simulink library "ConverterLibrary"  (R2026a)
settings: Solver=VariableStepAuto
undefined symbols (not defined in the file or in its folder): DiscIntNeverNeededParam, dspblkCoreblockFVToolHelper, gcbh, gridInverter
libraries: fl_lib x240, nesl_utility x221, ee_lib x208, slpidlib x28, eeGeneralControl x12, simulink x9, eeTransforms x4, simulink_extras x1, eePowerMeasurement x1
(part 1 of 30)
settings Model: Creator=vsolaise  LastModifiedBy=vsolaise

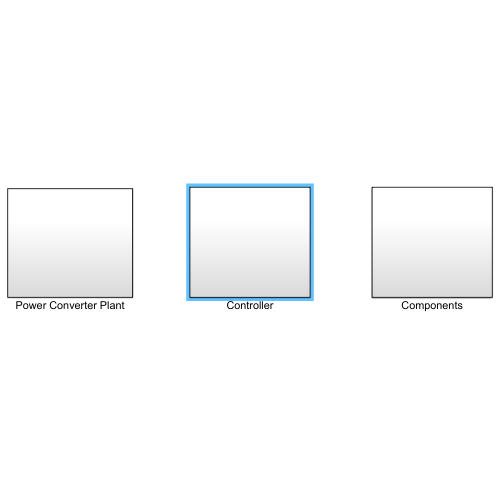
[thumbnail: Simulink's stored preview of the top-level diagram]
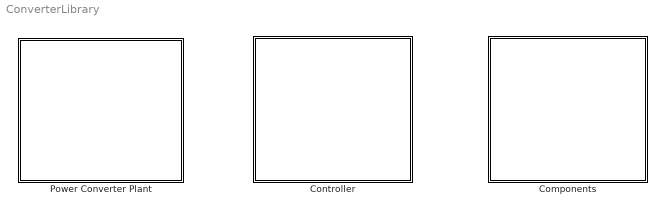
== system ConverterLibrary ==
  Components : Subsystem
  Controller : Subsystem
  Power Converter Plant : Subsystem

== system ConverterLibrary/Components ==
  Diode Model : Subsystem  mask(Diode thermal model){Tj_diode=[25, 125]+273.15, Tj_diode_unit=K, If_data=[.1, .2, .5, 1, 2, 4, 7, 10], If_data_unit=A, Vf_data=[.9, 1.15, 1.25, 1.5, 1.75, 2.17, 2.6, 2.85; .58, .68, .75, 1.1, 1.38, 1.77, 2.27, 2.7], Vf_data_unit=V, thermal_resistance=0.3, thermal_resistance_unit=K/W, thermal_mass=0.001, thermal_mass_unit=J/K, Tj0=300, Tj0_unit=K, diodeVf=0.8, diodeVf_unit=V, diodeRon=0.001, diodeRon_unit=Ohm, diodeGoff=1e-5, diodeGoff_unit=1/Ohm, Recovery_Loss_Flag=on, Tj_rec=[25, 125]+273.15, Tj_rec_unit=K, If_rec_data=[.1, .2, .5, 1, 2, 4, 7, 10], If_rec_data_unit=A, Erec_data=1e-6*[0.05 0.1 0.4 1 2.6 6 11.5 17.5; 0.1 0.2 0.8 2.1 5.2 12 23 35], Erec_data_unit=J, Vrec_ref=300, Vrec_ref_unit=V, Irec_min=1e-3, Irec_min_unit=A}
      mask prompts: Tj_diode "Junction temperature vector, Tj"; If_data "Forward current vector, If"; Vf_data "Forward voltage, Vf(Tj,If)"; thermal_resistance "Junction-case resistance"; thermal_mass "Junction thermal mass"; Tj0 "Initial temperature"; diodeVf "Forward voltage, Vf"; diodeRon "On-state resistance, Ron"; diodeGoff "Off-state conductance, Goff"; Recovery_Loss_Flag "Include reverse recovery loss"; Tj_rec "Junction temperature vector, Tj"; If_rec_data "Forward current vector before commutation, If"; Erec_data "Reverse recovery energy, Erec(Tj,If)"; Vrec_ref "Voltage at which Erec was measured, Vref"; Irec_min "Forward current below which the diode counts as off"
      mask help: This block implements a diode with a thermal port using a Simulink interface for better simulation performance. The electrical model is simple-fidelity; conduction loss is evaluated from the tabulated I-V curve and reverse recovery loss from a tabulated recovery energy, both in Simulink. Together they drive the junction temperature, which is applied back to the thermal port. Ports + and - are the electrical terminals; port A is the ambient (case) thermal port.
      mask init:
      | % Unit conversion - convert to internal units: V, A, Ohm, 1/Ohm, J, K, K/W, J/K
      | 
      | % Voltage (to V)
      | if strcmp(diodeVf_unit, 'mV'), diodeVf = diodeVf / 1000; end
      | if strcmp(Vf_data_unit, 'mV'), Vf_data = Vf_data / 1000; end
      | if strcmp(Vrec_ref_unit, 'kV'), Vrec_ref = Vrec_ref * 1000; end
      | 
      | % Current (to A)
      | if strcmp(If_data_unit, 'mA'), If_data = If_data / 1000; end
      | if strcmp(If_rec_data_unit, 'mA'), If_rec_data = If_rec_data / 1000; end
      | if strcmp(Irec_min_unit, 'mA'), Irec_min = Irec_min / 1000; end
      | 
      | % Resistance and conductance (to Ohm and 1/Ohm; S is identical to 1/Ohm)
      | if strcmp(diodeRon_unit, 'mOhm'), diodeRon = diodeRon / 1000; end
      | if strcmp(diodeGoff_unit, 'mS'), diodeGoff = diodeGoff / 1000; end
      | 
      | % Energy (to J)
      | if strcmp(Erec_data_unit, 'mJ'), Erec_data = Erec_data / 1000; end
      | if strcmp(Erec_data_unit, 'uJ'), Erec_data = Erec_data / 1e6; end
      | 
      | % Temperature (to K)
      | if strcmp(Tj_diode_unit, 'degC'), Tj_diode = Tj_diode + 273.15; end
      | if strcmp(Tj_rec_unit, 'degC'), Tj_rec = Tj_rec + 273.15; end
      | if strcmp(Tj0_unit, 'degC'), Tj0 = Tj0 + 273.15; end
      | 
      | % Thermal mass (to J/K)
      | if strcmp(thermal_mass_unit, 'kJ/K'), thermal_mass = thermal_mass * 1000; end
      | 
      | % Reverse recovery on or off. Folded into the Recovery step gain, so clearing
      | % the box removes the contribution rather than scaling it by something small.
      | if strcmp(get_param(gcb, 'Recovery_Loss_Flag'), 'on')
      |     RecoveryLossFlag = 1;
      | else
      |     RecoveryLossFlag = 0;
      | end
      mask Help: web('DiodeModel.html')
      mask TypeOptions Tj_diode_unit: K | degC
      mask TypeOptions If_data_unit: A | mA
      mask TypeOptions Vf_data_unit: V | mV
      mask TypeOptions thermal_resistance_unit: K/W | degC/W
      mask TypeOptions thermal_mass_unit: J/K | kJ/K
      mask TypeOptions Tj0_unit: K | degC
      mask TypeOptions diodeVf_unit: V | mV
      mask TypeOptions diodeRon_unit: Ohm | mOhm
      mask TypeOptions diodeGoff_unit: 1/Ohm | S | mS
      mask TypeOptions Tj_rec_unit: K | degC
      mask TypeOptions If_rec_data_unit: A | mA
      mask TypeOptions Erec_data_unit: J | mJ | uJ
      mask TypeOptions Vrec_ref_unit: V | kV
      mask TypeOptions Irec_min_unit: A | mA
      mask DialogControl conduction Prompt: Diode electrical parameters
      mask DialogControl switching Prompt: Reverse recovery loss parameters
      mask DialogControl diodeConduction Prompt: Conduction loss (I-V curve)
      mask DialogControl thermal Prompt: Thermal parameters
      mask Display: image('diode_thermal.svg');
  IGBT Model : Subsystem  mask(IGBT thermal model){Vth=0.5, Vth_unit=V, Von_data=[ 0 1.1 1.3 1.45 1.75 2.25 2.7; 0 1 1.15 1.35 1.7 2.35 3 ], Von_data_unit=V, Tj=[ 298.15 398.15 ], Tj_unit=K, Iout_data=0.1*[ 0 10 50 100 200 400 600 ], Iout_data_unit=A, Iout_data_loss=0.1*[ 0 10 50 100 200 400 600 ], Iout_data_loss_unit=A, Tj_loss=[ 298.15 398.15 ], Tj_loss_unit=K, Eoff_data=0.1*[ 0 2.1e-4 1.07e-3 2.14e-3 4.29e-3 9.86e-3 1.714e-2; 0 4.3e-4 1.97e-3 3.86e-3 7.71e-3 1.543e-2 2.271e-2 ], Eoff_data_unit=J, Eon_data=0.1*[ 0 2.9e-4 1.43e-3 2.86e-3 5.71e-3 1.314e-2 2.286e-2; 0 5.7e-4 2.63e-3 5.14e-3 1.029e-2 2.057e-2 3.029e-2 ], Eon_data_unit=J, Voff=300, Voff_unit=V, Soft_Switching_Flag=on, Tj_diode=[25, 125]+273.15, Tj_diode_unit=K, If_data=[.1, .2, .5, 1, 2, 4, 7, 10], If_data_unit=A, Vf_data=[.9, 1.15, 1.25, 1.5, 1.75, 2.17, 2.6, 2.85; .58, .68, .75, 1.1, 1.38, 1.77, 2.27, 2.7], Vf_data_unit=V, thermal_resistance=0.3, thermal_resistance_unit=K/W, thermal_mass=0.001, thermal_mass_unit=J/K, Tj0=300, Tj0_unit=K, VfIGBT=0.8, VfIGBT_unit=V, Ron=0.001, Ron_unit=Ohm, Goff=1e-5, Goff_unit=1/Ohm, diodeOption=Inbuilt diode, diodeVf=0.8, diodeVf_unit=V, diodeRon=0.001, diodeRon_unit=Ohm, diodeGoff=1e-5, diodeGoff_unit=1/Ohm}
      mask prompts: Vth "Threshold voltage"; Von_data "On-state voltage, Vce(Tj,Ice)"; Tj "Temperature vector, Tj"; Iout_data "Collector-emitter current vector, Ice"; Iout_data_loss "Collector-emitter current vector, Ice"; Tj_loss "Temperature vector, Tj"; Eoff_data "Switch-off loss, Eoff(Tj,Ids)"; Eon_data "Switch-on loss, Eon(Tj,Ids)"; Voff "Off-state voltage"; Soft_Switching_Flag "Soft-Switching Application"; Tj_diode "Temperature vector"; If_data "Current vector"; Vf_data "Diode voltage, Vf(Tj,Id)"; thermal_resistance "Junction-case resistance"; thermal_mass "Junction thermal mass"; Tj0 "Initial temperature"; VfIGBT "Forward voltage, Vf"; Ron "On-state resistance, Ron"; Goff "Off-state conductance, Goff"; diodeOption "Anti-parallel diode"; diodeVf "Diode forward voltage, Vf"; diodeRon "Diode on-state resistance, Ron"; diodeGoff "Diode off-state conductance, Goff"
      mask help: This block implements the IGBT (Ideal, Switching) with a thermal port using a Simulink interface for better simulation performance. Conduction, switching and anti-parallel diode losses are evaluated in Simulink and drive the junction temperature, which is applied back to the thermal port.
      mask init:
      | % Unit conversion - convert to internal units: V, A, Ohm, 1/Ohm, J, K, K/W, J/K
      | if strcmp(Vth_unit, 'mV'), Vth = Vth / 1000; end
      | if strcmp(VfIGBT_unit, 'mV'), VfIGBT = VfIGBT / 1000; end
      | if strcmp(Ron_unit, 'mOhm'), Ron = Ron / 1000; end
      | if strcmp(Goff_unit, 'mS'), Goff = Goff / 1000; end
      | if strcmp(Von_data_unit, 'mV'), Von_data = Von_data / 1000; end
      | if strcmp(Voff_unit, 'kV'), Voff = Voff * 1000; end
      | if strcmp(diodeVf_unit, 'mV'), diodeVf = diodeVf / 1000; end
      | if strcmp(diodeRon_unit, 'mOhm'), diodeRon = diodeRon / 1000; end
      | if strcmp(diodeGoff_unit, 'mS'), diodeGoff = diodeGoff / 1000; end
      | if strcmp(Vf_data_unit, 'mV'), Vf_data = Vf_data / 1000; end
      | if strcmp(Iout_data_unit, 'mA'), Iout_data = Iout_data / 1000; end
      | if strcmp(Iout_data_loss_unit, 'mA'), Iout_data_loss = Iout_data_loss / 1000; end
      | if strcmp(If_data_unit, 'mA'), If_data = If_data / 1000; end
      | if strcmp(Eoff_data_unit, 'mJ'), Eoff_data = Eoff_data / 1000; end
      | if strcmp(Eoff_data_unit, 'uJ'), Eoff_data = Eoff_data / 1e6; end
      | if strcmp(Eon_data_unit, 'mJ'), Eon_data = Eon_data / 1000; end
      | if strcmp(Eon_data_unit, 'uJ'), Eon_data = Eon_data / 1e6; end
      | if strcmp(Tj_unit, 'degC'), Tj = Tj + 273.15; end
      | if strcmp(Tj_loss_unit, 'degC'), Tj_loss = Tj_loss + 273.15; end
      | if strcmp(Tj_diode_unit, 'degC'), Tj_diode = Tj_diode + 273.15; end
      | if strcmp(Tj0_unit, 'degC'), Tj0 = Tj0 + 273.15; end
      | if strcmp(thermal_mass_unit, 'kJ/K'), thermal_mass = thermal_mass * 1000; end
      | 
      | % Off-state leakage loss: the IGBT, plus the anti-parallel diode when it is inbuilt.
      | if strcmp(get_param(gcb, 'diodeOption'), 'Inbuilt diode')
      |     leakageConductance = Goff + diodeGoff;
      | else
      |     leakageConductance = Goff;
      | end
      | 
      | % Hard- versus soft-switching sampling, consumed inside the Thermal model.
      | currentStatus = get_param(gcb, 'Soft_Switching_Flag');
      | if strcmp(currentStatus, 'on')
      |     SwitchLossFlag = 1;
      | else
      |     SwitchLossFlag = 0;
      | end
      | 
      | % Apply the anti-parallel diode option: variant choice plus parameter visibility.
      | selectIGBTModelDiodeOption(gcb);
      mask Help: web('IGBTModel.html')
      mask TypeOptions Vth_unit: V | mV
      mask TypeOptions Von_data_unit: V | mV
      mask TypeOptions Tj_unit: K | degC
      mask TypeOptions Iout_data_unit: A | mA
      mask TypeOptions Iout_data_loss_unit: A | mA
      mask TypeOptions Tj_loss_unit: K | degC
      mask TypeOptions Eoff_data_unit: J | mJ | uJ
      mask TypeOptions Eon_data_unit: J | mJ | uJ
      mask TypeOptions Voff_unit: V | kV
      mask Callback Soft_Switching_Flag:
      | currentStatus = get_param(gcb, 'Soft_Switching_Flag');
      | if strcmp(currentStatus, 'on')
      |     SwitchLossFlag = 1;
      | else
      |     SwitchLossFlag = 0;
      | end
      mask TypeOptions Tj_diode_unit: K | degC
      mask TypeOptions If_data_unit: A | mA
      mask TypeOptions Vf_data_unit: V | mV
      mask TypeOptions thermal_resistance_unit: K/W | degC/W
      mask TypeOptions thermal_mass_unit: J/K | kJ/K
      mask TypeOptions Tj0_unit: K | degC
      mask TypeOptions VfIGBT_unit: V | mV
      mask TypeOptions Ron_unit: Ohm | mOhm
      mask TypeOptions Goff_unit: 1/Ohm | S | mS
      mask TypeOptions diodeOption: Inbuilt diode | External diode
      mask Callback diodeOption: selectIGBTModelDiodeOption(gcb);
      mask TypeOptions diodeVf_unit: V | mV
      mask TypeOptions diodeRon_unit: Ohm | mOhm
      mask TypeOptions diodeGoff_unit: 1/Ohm | S | mS
      mask DialogControl conduction Prompt: IGBT conduction parameters
      mask DialogControl switching Prompt: IGBT switching parameters
      mask DialogControl diodeConduction Prompt: Anti-parallel diode parameters
      mask DialogControl thermal Prompt: Thermal parameters
      mask Display: image('n_igbt_thermal.svg');
  MOSFET Model : Subsystem  mask(MOSFET thermal model){Vth=3.2, Vth_unit=V, Von_data=[-3.075 -1.321 -0.5334 -0.2017 -5.735e-2 0 5.654e-2 0.1988 0.6074 1.756 5.672; -4.404 -1.709 -0.657 -0.2346 -0.0667 0 6.456e-2 0.227 0.6342 1.831 6.194; -4.759 -3.111 -1.191 -0.4253 -0.1209 0 0.1049 0.369 1.1 3.268 12.47; -5.366 -4.667 -1.787 -0.638 -0.1813 0 0.1573 0.5535 1.65 4.902 18.71], Von_data_unit=V, Tj=[-55 25 150 900], Tj_unit=degC, Iout_data=[-99.94 -39.11 -14.94 -5.333 -1.517 0 1.517 5.334 14.94 39.12 99.97], Iout_data_unit=A, Iout_data_loss=[0 16.04 32.08 48.12 64.15 80.19], Iout_data_loss_unit=A, Tj_loss=[-55 25 150 900 1000], Tj_loss_unit=degC, Eoff_data=[0 1.079e-4 2.792e-4 6.058e-4 1.107e-3 1.708e-3; 0 1.046e-4 2.706e-4 5.872e-4 1.073e-3 1.655e-3; 0 1.303e-4 3.368e-4 7.31e-4 1.336e-3 2.061e-3; 0 1.433e-4 3.705e-4 8.041e-4 1.47e-3 2.267e-3; 0 1.433e-4 3.705e-4 8.041e-4 1.47e-3 2.267e-3], Eoff_data_unit=J, Eon_data=[0 2.53e-4 7.404e-4 1.481e-3 2.418e-3 3.535e-3; 0 2.341e-4 6.85e-4 1.37e-3 2.237e-3 3.27e-3; 0 2.172e-4 6.356e-4 1.272e-3 2.076e-3 3.035e-3; 0 1.955e-4 5.72e-4 1.145e-3 1.868e-3 2.732e-3; 0 1.955e-4 5.72e-4 1.145e-3 1.868e-3 2.732e-3], Eon_data_unit=J, Voff=800, Voff_unit=V, Soft_Switching_Flag=on, Tj_diode=[-55 25 150 900 1000], Tj_diode_unit=degC, If_data=[0 1.516 5.33 14.93 39.07 99.82], If_data_unit=A, Vf_data=[0 3.294 3.769 4.385 5.249 6.672; 0 2.997 3.415 3.921 4.714 5.992; 0 2.624 2.988 3.498 4.274 5.6; 0 2.362 2.689 3.148 3.847 5.04; 0 2.362 2.689 3.148 3.847 5.04], Vf_data_unit=V, thermal_resistance=0.001, thermal_resistance_unit=K/W, thermal_mass=0.01, thermal_mass_unit=J/K, Tj0=25, Tj0_unit=degC, Goff=1e-5, Goff_unit=S, Rds=0.044, Rds_unit=Ohm, GdsOff=8.3333e-13, GdsOff_unit=S}
      mask prompts: Vth "Threshold voltage"; Von_data "On-state voltage, Vdson(Tj,Ids)"; Tj "Temperature vector, Tj"; Iout_data "Drain-source vector, Ids"; Iout_data_loss "Drain-source current vector, Ids"; Tj_loss "Temperature vector, Tj"; Eoff_data "Switch-off loss, Eoff(Tj,Ids)"; Eon_data "Switch-on loss, Eon(Tj,Ids)"; Voff "Off-state voltage"; Soft_Switching_Flag "Soft-Switching Application"; Tj_diode "Temperature vector"; If_data "Current vector"; Vf_data "Diode voltage Vf(Tj,Id)"; thermal_resistance "Junction-case resistance"; thermal_mass "Junction thermal mass"; Tj0 "Initial temperature"; Goff "Diode off-state conductance"; Rds "On-state resistance"; GdsOff "Off-state conductance"
      mask help: This block implements the MOSFET (Ideal, Switching) with thermal ports using SimuLink interface for better simulation performance.
      mask init:
      | % Unit conversion - convert to internal units: V, A, J, K, K/W, J/K, S
      | 
      | % Voltage (to V)
      | if strcmp(Vth_unit, 'mV'), Vth = Vth / 1000; end
      | if strcmp(Von_data_unit, 'mV'), Von_data = Von_data / 1000; end
      | if strcmp(Voff_unit, 'kV'), Voff = Voff * 1000; end
      | if strcmp(Vf_data_unit, 'mV'), Vf_data = Vf_data / 1000; end
      | 
      | % Current (to A)
      | if strcmp(Iout_data_unit, 'mA'), Iout_data = Iout_data / 1000; end
      | if strcmp(Iout_data_loss_unit, 'mA'), Iout_data_loss = Iout_data_loss / 1000; end
      | if strcmp(If_data_unit, 'mA'), If_data = If_data / 1000; end
      | 
      | % Energy (to J)
      | if strcmp(Eoff_data_unit, 'mJ'), Eoff_data = Eoff_data / 1000; end
      | if strcmp(Eoff_data_unit, 'uJ'), Eoff_data = Eoff_data / 1e6; end
      | if strcmp(Eon_data_unit, 'mJ'), Eon_data = Eon_data / 1000; end
      | if strcmp(Eon_data_unit, 'uJ'), Eon_data = Eon_data / 1e6; end
      | 
      | % Temperature (to K)
      | if strcmp(Tj_unit, 'degC'), Tj = Tj + 273.15; end
      | if strcmp(Tj_loss_unit, 'degC'), Tj_loss = Tj_loss + 273.15; end
      | if strcmp(Tj_diode_unit, 'degC'), Tj_diode = Tj_diode + 273.15; end
      | if strcmp(Tj0_unit, 'degC'), Tj0 = Tj0 + 273.15; end
      | 
      | % Thermal mass (to J/K)
      | if strcmp(thermal_mass_unit, 'kJ/K'), thermal_mass = thermal_mass * 1000; end
      | 
      | % Resistance (to Ohm)
      | if strcmp(Rds_unit, 'mOhm'), Rds = Rds / 1000; end
      | 
      | % Off-state conductance (to S)
      | if strcmp(GdsOff_unit, 'mS'), GdsOff = GdsOff / 1000; end
      | if strcmp(GdsOff_unit, 'uS'), GdsOff = GdsOff / 1e6; end
      | 
      | % Conductance (to S)
      | if strcmp(Goff_unit, 'mS'), Goff = Goff / 1000; end
      | if strcmp(Goff_unit, 'uS'), Goff = Goff / 1e6; end
      | 
      | currentStatus = get_param(gcb, 'Soft_Switching_Flag');
      | 
      | if strcmp(currentStatus, 'on')
      |     SwitchLossFlag = 1;
      | else
      |     SwitchLossFlag = 0;
      | end
      mask Help: web('MOSFET_Thermal_Model.html')
      mask TypeOptions Vth_unit: V | mV
      mask TypeOptions Von_data_unit: V | mV
      mask TypeOptions Tj_unit: K | degC
      mask TypeOptions Iout_data_unit: A | mA
      mask TypeOptions Iout_data_loss_unit: A | mA
      mask TypeOptions Tj_loss_unit: K | degC
      mask TypeOptions Eoff_data_unit: J | mJ | uJ
      mask TypeOptions Eon_data_unit: J | mJ | uJ
      mask TypeOptions Voff_unit: V | kV
      mask Callback Soft_Switching_Flag:
      | currentStatus = get_param(gcb, 'Soft_Switching_Flag');
      | 
      | if strcmp(currentStatus, 'on')
      |     SwitchLossFlag = 1;
      | else
      |     SwitchLossFlag = 0;
      | end
      mask TypeOptions Tj_diode_unit: K | degC
      mask TypeOptions If_data_unit: A | mA
      mask TypeOptions Vf_data_unit: V | mV
      mask TypeOptions thermal_resistance_unit: K/W | degC/W
      mask TypeOptions thermal_mass_unit: J/K | kJ/K
      mask TypeOptions Tj0_unit: K | degC
      mask TypeOptions Goff_unit: S | mS | uS
      mask TypeOptions Rds_unit: Ohm | mOhm
      mask TypeOptions GdsOff_unit: S | mS | uS
      mask DialogControl conduction Prompt: MOSFET Conduction parameters
      mask DialogControl switching Prompt: MOSFET switching parameters
      mask DialogControl diodeConduction Prompt: Diode conduction parameters
      mask DialogControl thermal Prompt: Thermal parameters
      mask Display: image('n_mosfet_thermal.svg');

== system ConverterLibrary/Controller ==
  Inverter-Based Resources : Subsystem
  Non-Isolated DC-DC Converters : Subsystem
  PWM Generators : Subsystem  AncestorBlock=ConverterLibrary/Controller/Non-Isolated DC-DC Converters
  Power Factor Correction Converters : Subsystem
  Soft-Switching Converters : Subsystem

== system ConverterLibrary/Power Converter Plant ==
  Non-Isolated DC-DC Converters : Subsystem
  Power Factor Correction Converters : Subsystem
  Soft-Switching Converters : Subsystem

== system ConverterLibrary/Components/Diode Model ==
  Diode : fl_lib/Electrical/Electrical Elements/Diode  Vf=diodeVf V  Ron=diodeRon Ohm  Goff=diodeGoff 1/Ohm  i_specify=off  i_priority=None  i=0 A  i_nominal_specify=off  i_nominal_value=1  i_nominal_unit=A  v_specify=off  v_priority=None  v=0 V  v_nominal_specify=off  v_nominal_value=1  v_nominal_unit=V
  Probe : SimscapeProbe  BoundBlock=5595  Variables="{\"i\":{\"Probing\":\"ON\"},\"v\":{\"Probing\":\"ON\"}}"
  Terminator : Terminator
  Thermal model : Subsystem
  + : PMIOPort  Side=Left
  - : PMIOPort  Port=2  Side=Right
  A : PMIOPort  Port=3  Side=Right
  wires:
  Thermal model/1(Tj) -> Terminator/1
  Probe/1 -> Thermal model/1(iD)
  Probe/2 -> Thermal model/2(vD)
  connections:
  A/RConn1 -- Thermal model/RConn1
  +/RConn1 -- Diode/LConn1
  -/RConn1 -- Diode/RConn1

== system ConverterLibrary/Components/IGBT Model ==
  Antiparallel Diode : Subsystem  Variant=on  VariantControlMode=label  LabelModeActiveChoice=InbuiltDiode
  Constant : Constant  Value=SwitchLossFlag
  IGBT : ee_lib/Semiconductors & Converters/IGBT (Ideal, Switching)  port_option=ee.enum.controlport.ps  Vf=VfIGBT V  Ron=Ron Ohm  Goff=Goff 1/Ohm  Vth=Vth V  diode_param=ee.enum.semiconductors.protectionDiode.external  diode_Vf=0.8 V  diode_Ron=0.001 Ohm  diode_Goff=1e-5 1/Ohm  diode_C=50e-9 F  diode_iRM=-235 A  diode_iF=300 A  diode_idot=-50 A/us  diode_trr_param=ee.enum.converters.diodeReverseParam.trr_factor  diode_trr_factor=3  diode_trr=15 us  diode_Qrr=1500 s*uA  ice_specify=off  ice_priority=None  ice=0 A  ice_nominal_specify=off  ice_nominal_value=1  ice_nominal_unit=A  vce_specify=off  vce_priority=None  vce=0 V  vce_nominal_specify=off  vce_nominal_value=1  vce_nominal_unit=V  vge_specify=off  vge_priority=None  vge=0 V  vge_nominal_specify=off  vge_nominal_value=1  vge_nominal_unit=V  thermal_loss_option=ee.enum.converters.thermalLossOption.constantvalues  Von_data=[0, .1, .6, .8, 1, 1.3, 1.6, 2, 2.4; 0, .1, .7, 1, 1.2, 1.5, 1.9, 2.4, 2.8] V  Tj=[298.15, 398.15] K  Iout_data=[0, .1, 1, 5, 10, 20, 40, 70, 100] A  tabulateWithVce=false  Eon_data=[0, .0024, .024, .12, .2, .48, 1.04, 2.16, 3.24; 0, .003, .03, .15, .25, .6, 1.3, 2.7, 4.05] * 1e-3 J  Eoff_data=[0, .0007, .0066, .033, .066, .17, .33, .83, 1.5; 0, .001, .01, .05, .1, .25, .5, 1.2, 2.2] * 1e-3 J  Eon_data_3D=[zeros(2, 9, 3)] J  Eoff_data_3D=[zeros(2, 9, 3)] J  Tj_loss=[298.15, 398.15] K  Iout_data_loss=[0, .1, 1, 5, 10, 20, 40, 70, 100] A  Vce_loss=[0, 150, 300] V  Eon_scalar=22.86e-3 J  Eoff_scalar=17.14e-3 J  Voff=300 V  Iout_scalar=600 A  useCurrentFromPreviousCycle=false  useVoltageFromPreviousCycle=false  diodeModelType=ee.enum.converters.diodeModelType.pwl  diodeTableType=ee.enum.diode.tableType.IfMat  diode_ReverseIVType=ee.enum.diode.diodeReverseIV.constant  diode_IfMat=[.07, .12, .19, 1.75, 4.24, 7.32, 11.2; .16, .3, .72, 2.14, 4.02, 6.35, 9.12] A  diode_VfMat=[.9, 1.15, 1.25, 1.5, 1.75, 2.17, 2.6, 2.85; .58, .68, .75, 1.1, 1.38, 1.77, 2.27, 2.7] V  diode_TjVec=[25, 125] degC  diode_VfVec=[.5, .7, .9, 1.3, 1.7, 2.1, 2.5] V  diode_IfVec=[.1, .2, .5, 1, 2, 4, 7, 10] A  diode_IrMat=[1e-06, 2e-06, 5e-06, 1e-05, 2.5e-05, 5e-05, .0001; 2e-06, 5e-06, 1e-05, 4e-05, 8e-05, .0002, .0005] A  diode_VrMat=[10, 100, 200, 250, 300, 325, 350; 10, 70, 160, 220, 270, 300, 320] V  diode_VrVec=[10, 20, 40, 50, 70, 80, 100] V  diode_IrVec=[1e-06, 2e-06, 5e-06, 1e-05, 2e-05, 5e-05, .0001] A  diode_Vr=-600 V  diode_Ls=150 nH  diode_Erec=0.03 J  diode_rec_loss_model=ee.enum.diode.reverseRecoveryModelTabulateUpTo3D.fixed  diode_ErecVal=0 J  diode_scaleWithIandV=true  diode_ErecMat=zeros(2, 3) J  diodeErecMat3D=zeros(2, 3, 2) J  diode_TjrecVec=[298.15, 398.15] K  diode_IfrecVec=[.1, 1, 10] A  diodeVrecVec=[0, 100] V  diode_IrecVal=10 A  diode_VrecVal=10 V  diode_tFilter=1 / 1000 / 100 s  separateThermalPortForDiode=false  thermal_network_parameterization=ee.enum.thermalNetworkTopology.external  Rth=[.08, .5] K/W  Rth_Cauer=[.08, .1, .5] K/W  Rth_Foster=[.08, .14, .22, .16] K/W  thermal_mass_parameterization=ee.enum.thermalNetwork.timeconstant  thermal_mass=[.01, .5] J/K  thermal_mass_Cauer=[.01, .1, .5] J/K  thermal_mass_Foster=[.001, .005, .05, .5] J/K  thermal_time_constant=[.001, .2] s  thermal_time_constant_Cauer=[.001, .1, .2] s  thermal_time_constant_Foster=[7e-05, .0007, .01, .08] s  thermal_mass_initial_temperatures=[25, 25] degC  thermal_mass_initial_temperatures_Cauer=[25, 25, 25] degC  junction_thermal_mass=0.01 J/K  Tvec_initial_Foster=[25, 25, 25, 25] degC  RthDiode=[.03, .2] K/W  RthCauerDiode=[.03, .1, .2] K/W  RthFosterDiode=[.03, .2] K/W  thermalMassDiode=[3, 25] J/K  thermalMassCauerDiode=[3, 10, 25] J/K  thermalMassFosterDiode=[33, 50] J/K  thermalTauDiode=[.1, 5] s  thermalTauCauerDiode=[.1, 1, 5] s  thermalTauFosterDiode=[1, 10] s  thermalMassInitTempDiode=[25, 25] degC  thermalMassInitTempCauerDiode=[25, 25, 25] degC  junctionthermalMassDiode=0.1 J/K  TVecInitialFosterDiode=[25, 25, 25, 25] degC  no_thermal_network=ee.enum.enable.yes  IGBT_junction_temperature_specify=off  IGBT_junction_temperature_priority=None  IGBT_junction_temperature=25 degC  IGBT_junction_temperature_nominal_specify=off  IGBT_junction_temperature_nominal_value=1  IGBT_junction_temperature_nominal_unit=degC  diode_junction_temperature_specify=off  diode_junction_temperature_priority=None  diode_junction_temperature=25 degC  diode_junction_temperature_nominal_specify=off  diode_junction_temperature_nominal_value=1  diode_junction_temperature_nominal_unit=degC  Qj_specify=off  Qj_priority=None  Qj=0 W  Qj_nominal_specify=off  Qj_nominal_value=1  Qj_nominal_unit=W  accumulatedSwitchingLosses_specify=off  accumulatedSwitchingLosses_priority=None  accumulatedSwitchingLosses=0 J
  PS Constant : fl_lib/Physical Signals/Sources/PS Constant  constant=-1
  PS Constant1 : fl_lib/Physical Signals/Sources/PS Constant  constant=1
  PS Switch : fl_lib/Physical Signals/Nonlinear Operators/PS Switch  Threshold=Vth  ZeroCross=true
  PS-Simulink Converter : nesl_utility/PS-Simulink Converter  PhysicalDomain=network_engine_domain  SubClassName=ps_output  LeftPortType=input  RightPortType=output  PseudoPeriodic=off  Frequencies=[]  VectorFormat=inherit  Unit=inherit  AffineConversion=off
  Probe : SimscapeProbe  BoundBlock=5831  Variables="{\"ice\":{\"Probing\":\"ON\"},\"vce\":{\"Probing\":\"ON\"}}"
  Terminator : Terminator
  Thermal model : Subsystem
  G : PMIOPort  Side=Left
  C : PMIOPort  Port=2  Side=Right
  E : PMIOPort  Port=3  Side=Right
  A : PMIOPort  Port=4  Side=Left
  wires:
  PS-Simulink Converter/1 -> Thermal model/1(state)
  Probe/1 -> Thermal model/2(ice)
  Probe/2 -> Thermal model/3(vce)
  Antiparallel Diode/1(Id) -> Thermal model/4(Id)
  Constant/1 -> Thermal model/5(SwitchFlag)
  Thermal model/1(Tj) -> Terminator/1
  connections:
  C/RConn1 -- IGBT/RConn1 -- Antiparallel Diode/LConn1
  E/RConn1 -- IGBT/RConn2 -- Antiparallel Diode/LConn2
  G/RConn1 -- IGBT/LConn1 -- PS Switch/LConn2
  PS-Simulink Converter/LConn1 -- PS Switch/RConn1
  PS Constant/RConn1 -- PS Switch/LConn1
  PS Constant1/RConn1 -- PS Switch/LConn3
  Thermal model/RConn1 -- A/RConn1

== system ConverterLibrary/Components/MOSFET Model ==
  Constant : Constant  Value=SwitchLossFlag
  Diode : fl_lib/Electrical/Electrical Elements/Diode  Vf=0.01 V  Ron=1e-4 Ohm  Goff=Goff 1/Ohm  i_specify=off  i_priority=None  i=0 A  i_nominal_specify=off  i_nominal_value=1  i_nominal_unit=A  v_specify=off  v_priority=None  v=0 V  v_nominal_specify=off  v_nominal_value=1  v_nominal_unit=V
  "MOSFET (Ideal, Switching)1" : ee_lib/Semiconductors & Converters/MOSFET (Ideal, Switching)  port_option=ee.enum.controlport.ps  Rds=Rds Ohm  Goff=GdsOff 1/Ohm  Vth=Vth V  diode_param=ee.enum.semiconductors.protectionDiode.external  diode_Vf=0.8 V  diode_Ron=0.001 Ohm  diode_Goff=1e-5 1/Ohm  diode_C=50e-9 F  diode_iRM=-235 A  diode_iF=300 A  diode_idot=-50 A/us  diode_trr_param=ee.enum.converters.diodeReverseParam.trr_factor  diode_trr_factor=3  diode_trr=15 us  diode_Qrr=1500 s*uA  ids_specify=off  ids_priority=None  ids=0 A  ids_nominal_specify=off  ids_nominal_value=1  ids_nominal_unit=A  vds_specify=off  vds_priority=None  vds=0 V  vds_nominal_specify=off  vds_nominal_value=1  vds_nominal_unit=V  vgs_specify=off  vgs_priority=None  vgs=0 V  vgs_nominal_specify=off  vgs_nominal_value=1  vgs_nominal_unit=V  thermal_loss_option=ee.enum.converters.thermalLossOption.constantvalues  Von_data=[0, 1.8, 3.2, 6, 10, 16; 0, 2, 5.5, 9.5, 15, 25] V  Tj=[298.15, 448.15] K  Iout_data=[0, 20, 40, 60, 80, 100] A  tabulateWithVds=false  Eon_data=[0, 55.04, 124.57, 235.53, 362.12; 0, 71.25, 161.25, 304.88, 468.75] * 1e-6 J  Eoff_data=[0, 18, 30, 56.1, 76.5; 0, 22.5, 37.5, 70.13, 95.63] * 1e-6 J  Eon_data_3D=[zeros(2, 5, 3)] J  Eoff_data_3D=[zeros(2, 5, 3)] J  Tj_loss=[298.15, 448.15] K  Iout_data_loss=[0, 10, 20, 30, 40] A  Vds_loss=[0, 150, 300] V  Eon_scalar=22.86e-3 J  Eoff_scalar=17.14e-3 J  Voff=300 V  Iout_scalar=600 A  useCurrentFromPreviousCycle=false  useVoltageFromPreviousCycle=false  diodeModelType=ee.enum.converters.diodeModelType.pwl  diodeTableType=ee.enum.diode.tableType.IfMat  diode_ReverseIVType=ee.enum.diode.diodeReverseIV.constant  diode_IfMat=[.07, .12, .19, 1.75, 4.24, 7.32, 11.2; .16, .3, .72, 2.14, 4.02, 6.35, 9.12] A  diode_VfMat=[.9, 1.15, 1.25, 1.5, 1.75, 2.17, 2.6, 2.85; .58, .68, .75, 1.1, 1.38, 1.77, 2.27, 2.7] V  diode_TjVec=[25, 125] degC  diode_VfVec=[.5, .7, .9, 1.3, 1.7, 2.1, 2.5] V  diode_IfVec=[.1, .2, .5, 1, 2, 4, 7, 10] A  diode_IrMat=[1e-06, 2e-06, 5e-06, 1e-05, 2.5e-05, 5e-05, .0001; 2e-06, 5e-06, 1e-05, 4e-05, 8e-05, .0002, .0005] A  diode_VrMat=[10, 100, 200, 250, 300, 325, 350; 10, 70, 160, 220, 270, 300, 320] V  diode_VrVec=[10, 20, 40, 50, 70, 80, 100] V  diode_IrVec=[1e-06, 2e-06, 5e-06, 1e-05, 2e-05, 5e-05, .0001] A  diode_Vr=-600 V  diode_Ls=150 nH  diode_Erec=0.03 J  diode_rec_loss_model=ee.enum.diode.reverseRecoveryModel.fixed  diode_ErecVal=0 J  diode_scaleWithIandV=true  diode_ErecMat=zeros(2, 3) J  diodeErecMat3D=zeros(2, 3, 2) J  diode_TjrecVec=[298.15, 398.15] K  diode_IfrecVec=[.1, 1, 10] A  diodeVrecVec=[0, 100] V  diode_IrecVal=10 A  diode_VrecVal=10 V  diode_tFilter=1 / 1000 / 100 s  separateThermalPortForDiode=false  thermal_network_parameterization=ee.enum.thermalNetworkTopology.external  Rth=[.03, .2] K/W  Rth_Cauer=[.03, .1, .2] K/W  Rth_Foster=[.08, .14, .22, .16] K/W  thermal_mass_parameterization=ee.enum.thermalNetwork.timeconstant  thermal_mass=[3, 25] J/K  thermal_mass_Cauer=[3, 10, 25] J/K  thermal_mass_Foster=[.001, .005, .05, .5] J/K  thermal_time_constant=[.1, 5] s  thermal_time_constant_Cauer=[.1, 1, 5] s  thermal_time_constant_Foster=[7e-05, .0007, .01, .08] s  thermal_mass_initial_temperatures=[25, 25] degC  thermal_mass_initial_temperatures_Cauer=[25, 25, 25] degC  junction_thermal_mass=0.1 J/K  Tvec_initial_Foster=[25, 25, 25, 25] degC  RthDiode=[.03, .2] K/W  RthCauerDiode=[.03, .1, .2] K/W  RthFosterDiode=[.03, .2] K/W  thermalMassDiode=[3, 25] J/K  thermalMassCauerDiode=[3, 10, 25] J/K  thermalMassFosterDiode=[33, 50] J/K  thermalTauDiode=[.1, 5] s  thermalTauCauerDiode=[.1, 1, 5] s  thermalTauFosterDiode=[1, 10] s  thermalMassInitTempDiode=[25, 25] degC  thermalMassInitTempCauerDiode=[25, 25, 25] degC  junctionthermalMassDiode=0.1 J/K  TVecInitialFosterDiode=[25, 25, 25, 25] degC  no_thermal_network=0  mosfet_junction_temperature_specify=off  mosfet_junction_temperature_priority=None  mosfet_junction_temperature=25 degC  mosfet_junction_temperature_nominal_specify=off  mosfet_junction_temperature_nominal_value=1  mosfet_junction_temperature_nominal_unit=degC  diode_junction_temperature_specify=off  diode_junction_temperature_priority=None  diode_junction_temperature=25 degC  diode_junction_temperature_nominal_specify=off  diode_junction_temperature_nominal_value=1  diode_junction_temperature_nominal_unit=degC  Qj_specify=off  Qj_priority=None  Qj=0 W  Qj_nominal_specify=off  Qj_nominal_value=1  Qj_nominal_unit=W  accumulatedSwitchingLosses_specify=off  accumulatedSwitchingLosses_priority=None  accumulatedSwitchingLosses=0 J
  PS Constant : fl_lib/Physical Signals/Sources/PS Constant  constant=-1
  PS Constant1 : fl_lib/Physical Signals/Sources/PS Constant  constant=1
  PS Switch : fl_lib/Physical Signals/Nonlinear Operators/PS Switch  Threshold=Vth  ZeroCross=true
  PS-Simulink Converter : nesl_utility/PS-Simulink Converter  PhysicalDomain=network_engine_domain  SubClassName=ps_output  LeftPortType=input  RightPortType=output  PseudoPeriodic=off  Frequencies=[]  VectorFormat=inherit  Unit=inherit  AffineConversion=off
  Probe : SimscapeProbe  BoundBlock=11105  Variables="{\"ids\":{\"Probing\":\"ON\"},\"vds\":{\"Probing\":\"ON\"}}"
  Probe1 : SimscapeProbe  BoundBlock=11104  Variables="{\"i\":{\"Probing\":\"ON\"}}"
  SPST Switch : ee_lib/Switches & Breakers/SPST Switch  R_closed=1e-4 Ohm  G_open=1e-6 S  Threshold=0 V  Width=0 V  model_dynamics=0  t_on=1e-3 s  t_off=1e-3 s  initial_vT=0 V
  Terminator : Terminator
  Thermal model : Subsystem
  G : PMIOPort  Side=Left
  D : PMIOPort  Port=2  Side=Right
  S : PMIOPort  Port=3  Side=Right
  A : PMIOPort  Port=4  Side=Left
  wires:
  Constant/1 -> Thermal model/5(SwitchFlag)
  PS-Simulink Converter/1 -> Thermal model/1(state)
  Probe/2 -> Thermal model/3(vds)
  Probe/1 -> Thermal model/2(ids)
  Probe1/1 -> Thermal model/4(Id)
  Thermal model/1(Tj) -> Terminator/1
  connections:
  PS Constant1/RConn1 -- PS Switch/LConn3
  PS Constant/RConn1 -- PS Switch/LConn1
  PS-Simulink Converter/LConn1 -- SPST Switch/LConn1 -- PS Switch/RConn1
  SPST Switch/RConn1 -- Diode/RConn1
  PS Switch/LConn2 -- "MOSFET (Ideal, Switching)1"/LConn1 -- G/RConn1
  A/RConn1 -- Thermal model/RConn1
  "MOSFET (Ideal, Switching)1"/RConn2 -- Diode/LConn1 -- S/RConn1
  "MOSFET (Ideal, Switching)1"/RConn1 -- SPST Switch/LConn2 -- D/RConn1

== system ConverterLibrary/Controller/Inverter-Based Resources ==
  Grid-Forming Converter Controller : Subsystem  mask(Grid-Forming Controller){power=500e3, gridLineVoltage=415, powerFreq=50, dcBusVoltage=1100, measSampleTime=0.0001, powerControl=Virtual Synchronous Machine, activePowerSampleTime=0.0001, droopSlope=0.01, droopT1=0.005, droopT2=0.006, droopTC=0.015, vsmPmeasFilterTC=0.001, vsmFreqDroop=10, vsmInertiaTC=1, vsmDampingConst=1.056, dampingPowerMaxLimit=0.7, dampingPowerMinLimit=-0.6, freqMeasTimeConst=0.15, freqOption=Grid Frequency Measurement, voltreference=1, QVoltFilterTC=0.001, QVoltDroop=0.3, lowVoltageSupportGain=1.5, currentLimit=Virtual Impedance, maxSatCurrentLimit=1.4, maxVICurrentLimit=1.2, ctLimitVirtualImp=2.0625e-1, ctLimitXbyR=13.2, ctLimitDelayTime=0.001, currentSatTime=0.001, currentVITimeConst=0.001, modeTransferTime=10*gridInverter.controller.CurrentControlSampleTime, voltControlTs=0.0001, vdPGain=0.3, VdIGain=180, VdMaxCt=1.8, VdMinCt=-1.8, VqPGain=0.3, VqIGain=180, VqMaxCt=1.8, VqMinCt=-1.8, vdvqLPFTimeConst=0.005, currentControlTs=0.0001, filterInductance=1.0964e-4, IdPGain=1.5, IdIGain=10, IqPGain=1.5, IqIGain=10}
      mask prompts: power "Grid-forming converter power (VA)"; gridLineVoltage "Grid line voltage (V)"; powerFreq "Grid frequency (Hz)"; dcBusVoltage "DC bus voltage (V)"; measSampleTime "Measurement sample time (s)"; powerControl "Active Power Control"; activePowerSampleTime "Power controller sample time (s)"; droopSlope "Power droop slope (pu, Hz/W)"; droopT1 "Lead-Lag numerator time constant (s)"; droopT2 "Lead-Lag denominator time constant (s)"; droopTC "Filter cut-off time constant (s)"; vsmPmeasFilterTC "Power measurement filter time constant (s)"; vsmFreqDroop "Frequency droop (pu,  W/Hz)"; vsmInertiaTC "Inertia constant M (pu)"; vsmDampingConst "Damping constant (pu/Hz)"; dampingPowerMaxLimit "Damping power maximum limit (pu)"; dampingPowerMinLimit "Damping power minimum limit (pu)"; freqMeasTimeConst "Frequency measurement time constant (s)"; freqOption "Damping power frequency option"; voltreference "Voltage reference value (pu)"; QVoltFilterTC "Power measurement filter time constant (s)"; QVoltDroop "Voltage droop (pu, V/VAr)"; lowVoltageSupportGain "Low voltage support gain (pu, A/V)"; currentLimit "Current limiting method"; maxSatCurrentLimit "Maximum current saturation (pu)"; maxVICurrentLimit "Maximum virtual impedance current (pu)"; ctLimitVirtualImp "Virtual impedance coefficient (pu.Ohm/pu.A)"; ctLimitXbyR "Virtual X/R ratio"; ctLimitDelayTime "Maximum current delay time (s)"; currentSatTime "Current limiting run time (s)"; currentVITimeConst "Filter time constant (s)"; modeTransferTime "Mode transfer time (s)"; voltControlTs "Voltage controller sample time (s)"; vdPGain "Vd proportional gain"; VdIGain "Vd integral gain"; VdMaxCt "Vd maximum current limit (A)"; VdMinCt "Vd minimum current limit (A)"; VqPGain "Vq proportional gain"; VqIGain "Vq integral gain"; VqMaxCt "Vq maximum current limit (A)"; VqMinCt "Vq minimum current limit (A)"; vdvqLPFTimeConst "Voltage measurement filter time constant (s)"; currentControlTs "Current controller sample time (s)"; filterInductance "Filter inductance (H)"; IdPGain "Id proportional gain"; IdIGain "Id integral gain"; IqPGain "Iq proportional gain"; IqIGain "Iq integral gain"
      mask help: This block implements the grid forming controller with fault ride through capability. Input to the controller are active and reactive power reference in per unit and the sensed three-phase phase current in amphere and phase voltage in volts.
      mask init:
      | gfmControllerMaskInitialization(gcb);
      settings: CopyFcn="set_param(gcbh,\"LinkStatus\",\"none\");"
      mask Help: web("GFMController.html")
      mask TypeOptions powerControl: Virtual Synchronous Machine | Droop Control
      mask Callback powerControl: selectGFMActivePowerControl(gcb);
      mask TypeOptions freqOption: Grid Frequency Measurement | Constant Frequency Reference
      mask TypeOptions currentLimit: Virtual Impedance | Current Limiting | Virtual Impedance and Current Limiting
      mask Callback currentLimit: selectGFMFaultRideThroughMethod(gcb);
      mask DialogControl ParameterGroupVar Prompt: Grid-Forming Controller Parameters
      mask DialogControl GFMGroup Prompt: Grid-Forming Converter Specifications
      mask DialogControl Pcontrolgrp Prompt: Active Power Controller Parameters
      mask DialogControl QcontrolGrp Prompt: Reactive Power Controller Parameters
      mask DialogControl faultRideThroughGrp Prompt: Fault Ride-Through Parameters
      mask DialogControl voltControlgrp Prompt: Voltage Controller Parameters
      mask DialogControl Container15currentContGrp Prompt: Current Controller Parameters
      mask Display: image('$imagefile'); % Use "Edit Image" on toolstrip to change.

== system ConverterLibrary/Controller/Non-Isolated DC-DC Converters ==
  Non-Isolated DC-DC Controller : Subsystem  mask(Non-Isolated DCDC Cascaded Controller){modelOption=Synchronous Boost, loopStructure=Double loop, cntrlSelect=PI controller (Continuous), outputSelect=PWM Signal, VbaseIn=200, VbaseOut=400, Pbase=1500, dutyMax=0.95, dutyMin=0.02, Fsw=100000, Tdead=1e-07, Ts=1e-08, gateVoltageOn=15, gateVoltageOff=0, KpVoltage=38, KiVoltage=31415.9265, TsVoltage=0.0001, iRefMaxPu=1.5, iRefMinPu=0, softStartTime=0.004, KpCurrent=0.2566, KiCurrent=806.0999, TsCurrent=1e-05}
      mask prompts: modelOption "Topology"; loopStructure "Control structure"; cntrlSelect "Controller type"; outputSelect "Output signal"; VbaseIn "Input voltage base (V)"; VbaseOut "Output voltage base (V)"; Pbase "Power base (W)"; dutyMax "Maximum duty cycle"; dutyMin "Minimum duty cycle"; Fsw "Switching frequency (Hz)"; Tdead "Dead time (s)"; Ts "Sample time (s)"; gateVoltageOn "Gate ON voltage (V)"; gateVoltageOff "Gate OFF voltage (V)"; KpVoltage "Proportional gain (pu)"; KiVoltage "Integral gain (pu/s)"; TsVoltage "Sample time (s)"; iRefMaxPu "Maximum current reference (pu)"; iRefMinPu "Minimum current reference (pu)"; softStartTime "Soft-start time (s)"; KpCurrent "Proportional gain (pu)"; KiCurrent "Integral gain (pu/s)"; TsCurrent "Sample time (s)"
      mask help: Cascaded average-current-mode controller for the non-isolated DC-DC converter, covering all six plant topologies. An outer voltage loop commands the per-unit inductor current and an inner current loop trims the duty about a topology-based feedforward. Offers PI controllers in continuous or discrete form, with selectable duty cycle or PWM gate signal output.
      mask init:
      | % Topology family.
      | isSynchronous = any(strcmp(modelOption, ...
      |     {'Synchronous Buck', 'Synchronous Boost', 'Synchronous Buck-Boost'}));
      | isBuck = any(strcmp(modelOption, {'Buck', 'Synchronous Buck'}));
      | isBoost = any(strcmp(modelOption, {'Boost', 'Synchronous Boost'}));
      | 
      | % Feedforward duty at the nominal operating point.
      | if isBuck
      |     dutyNominal = VbaseOut/VbaseIn;
      | elseif isBoost
      |     dutyNominal = 1 - VbaseIn/VbaseOut;
      | else
      |     dutyNominal = VbaseOut/(VbaseIn + VbaseOut);
      | end
      | 
      | % Inductor current base: output current in a buck, input current in a boost, both in a buck-boost.
      | if isBuck
      |     IbaseL = Pbase/VbaseOut;
      | elseif isBoost
      |     IbaseL = Pbase/VbaseIn;
      | else
      |     IbaseL = Pbase/VbaseIn + Pbase/VbaseOut;
      | end
      | 
      | % Feedforward divisor floors, 5% of nominal, so the laws stay finite at startup.
      | voltageReferencePuMin = 0.05;
      | inputVoltagePuMin = 0.05*VbaseIn/VbaseOut;
      | 
      | % Soft-start ramp. A boost output starts at the input voltage through the body diode.
      | if isBoost
      |     referenceStartPu = VbaseIn/VbaseOut;
      | else
      |     referenceStartPu = 0;
      | end
      | referenceSlewRatePu = (1 - referenceStartPu)/max(softStartTime, eps);
      | 
      | % Modulator: second gate and dead time only for a synchronous leg.
      | gateIndices = 1:(1 + isSynchronous);
      | pwmDeadTime = Tdead*isSynchronous;
      | 
      | % Voltage controller limits: current reference in the double loop, duty trim in the single loop.
      | if strcmp(loopStructure, 'Double loop')
      |     voltageLimitUpper = iRefMaxPu;
      |     voltageLimitLower = iRefMinPu;
      | else
      |     voltageLimitUpper = dutyMax - dutyNominal;
      |     voltageLimitLower = dutyMin - dutyNominal;
      | end
      | voltageIntegratorInit = min(voltageLimitUpper, max(voltageLimitLower, 0));
      | 
      | % Current controller integrator backstop; the live clamp uses the external limits.
      | dutyTrimSpan = dutyMax - dutyMin;
      | 
      | nonIsolatedDCDCControllerMaskInit(gcb);
      mask Help: web('NonIsolatedDCDCController.html')
      mask TypeOptions modelOption: Buck | Synchronous Buck | Boost | Synchronous Boost | Buck-Boost | Synchronous Buck-Boost
      mask Callback modelOption: nonIsolatedDCDCControllerMaskInit(gcb);
      mask TypeOptions loopStructure: Single loop | Double loop
      mask Callback loopStructure: nonIsolatedDCDCControllerMaskInit(gcb);
      mask TypeOptions cntrlSelect: PI controller (Continuous) | PI controller (Discrete)
      mask Callback cntrlSelect: nonIsolatedDCDCControllerMaskInit(gcb);
      mask TypeOptions outputSelect: PWM Signal | Duty Cycle
      mask Callback outputSelect: nonIsolatedDCDCControllerMaskInit(gcb);
      mask DialogControl ConverterPanel Prompt: Converter and Modulator
      mask DialogControl VoltageLoopPanel Prompt: Voltage Controller
      mask DialogControl CurrentLoopPanel Prompt: Current Controller
